simulink model "UAV3_Energy_07"  (R2026b)
settings: Solver=FixedStepDiscrete  FixedStep=0.1
settings Model: Creator=Ivan  LastModifiedBy=Ivan

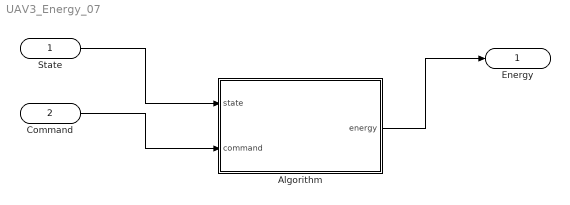
== system UAV3_Energy_07 ==
  State : Inport  OutDataTypeStr=double  PortDimensions=[5 1]
  Command : Inport  Port=2  OutDataTypeStr=double  PortDimensions=[2 1]
  Algorithm : MATLAB Function  TreatAsAtomicUnit=on
  Energy : Outport
  wires:
  State/1 -> Algorithm/1(state)
  Command/1 -> Algorithm/2(command)
  Algorithm/1(energy) -> Energy/1

== matlab function UAV3_Energy_07/Algorithm ==
  data: state input; energy output; command input
function energy = v3_energy(state,command)
%V3_ENERGY Lightweight percent-per-second battery model.
% energy=[drainPercentPerSecond;stateBattery;lowFlag].
%#codegen
speed=sqrt(sum(state(3:4).^2));
accel=sqrt(sum(command.^2));
drain=0.08+0.012*speed+0.002*accel;
energy=[drain;state(5);double(state(5)<=20.0)];
end
